simulink library "quadcopter_lib"  (R2018b)
settings: Solver=VariableStepAuto  StartTime=0.0  StopTime=10.0  RelTol=1e-3
undefined symbols (not defined in the file or in its folder): copter, grnd, IC, pos_ref
libraries: actuators_lib x1, ground_lib x1, multicopter_aerodynamics_simple_lib x1, quadcopter_propulsion_lib x1, rigidBody_lib x1
settings Model: Creator=Ybeyer  LastModifiedBy=yannic
settings SFSimCC: SimUseLocalCustomCode=off
settings RTWCC: RTWUseLocalCustomCode=off
settings CodeAppCC: StateflowObjectComments=on

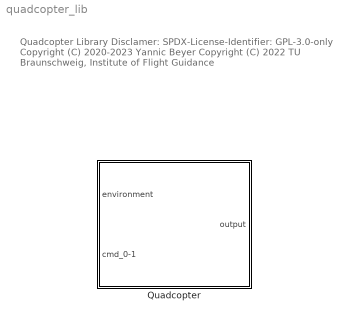
== system quadcopter_lib ==
  note: Quadcopter Library
      |
      | Disclamer:
      | SPDX-License-Identifier: GPL-3.0-only
      |
      | Copyright (C) 2020-2023 Yannic Beyer
      | Copyright (C) 2022 TU Braunschweig, Institute of Flight Guidance
  Quadcopter : Subsystem  mask{copter_=copter, IC_=IC, grnd_=grnd}
      mask prompts: copter_ "copter parameters struct"; IC_ "initial conditions struct"; grnd_ "ground contact parameters struct"
      mask DialogControl DescGroupVar Prompt: Quadcopter
      mask DialogControl DescTextVar Prompt: Standard rigid-body quadcopter model with map-based propellers and simple aerodynamics model for the frame

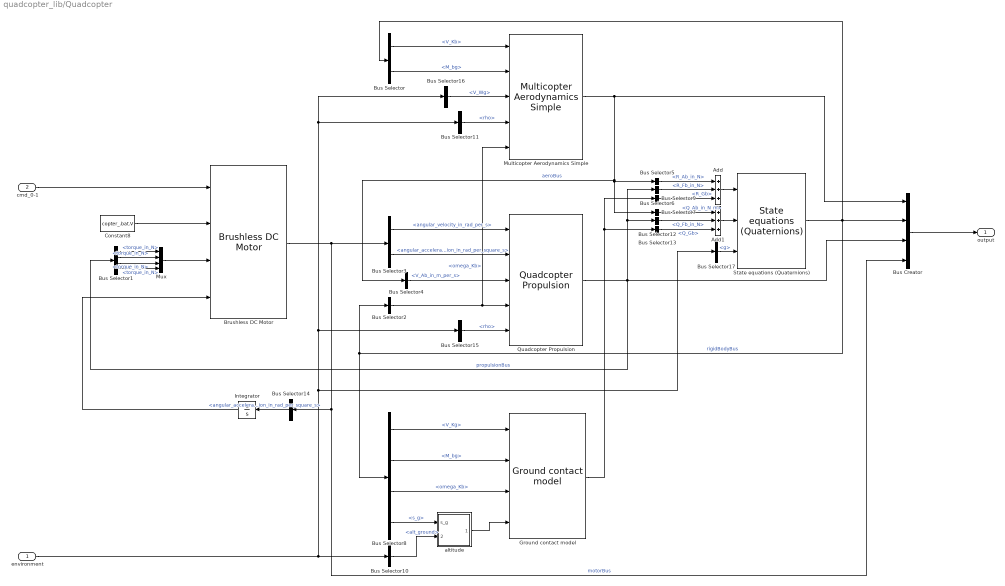
== system quadcopter_lib/Quadcopter ==
  environment : Inport  OutDataTypeStr=Bus: envirBus
  cmd_0-1 : Inport  Port=2  OutDataTypeStr=double  PortDimensions=4
  Add : Sum  Inputs=+++
  Add1 : Sum  Inputs=+++
  Brushless DC Motor : actuators_lib/Brushless DC Motor  K_T=copter_.motor.KT  J_prop=copter_.prop.I  R_i=copter_.motor.R  IC_omega=IC_.omega_mot  omega_max=Inf  omega_min=0
      settings: SourceProductName=LADAC
  Bus Creator : BusCreator  Inputs=4
  Bus Selector : BusSelector  OutputSignals=V_Kb,M_bg
  Bus Selector1 : BusSelector  OutputSignals=propeller_1.torque_in_N,propeller_2.torque_in_N,propeller_3.torque_in_N,propeller_4.torque_in_N
  Bus Selector10 : BusSelector  OutputSignals=alt_ground
  Bus Selector11 : BusSelector  OutputSignals=atmosphere.rho
  Bus Selector12 : BusSelector  OutputSignals=Q_Fb_in_N
  Bus Selector13 : BusSelector  OutputSignals=forces_and_moments.Q_Gb
  Bus Selector14 : BusSelector  OutputSignals=angular_acceleration_in_rad_per_square_s
  Bus Selector15 : BusSelector  OutputSignals=atmosphere.rho
  Bus Selector16 : BusSelector  OutputSignals=wind.V_Wg
  Bus Selector17 : BusSelector  OutputSignals=g
  Bus Selector2 : BusSelector  OutputSignals=omega_Kb
  Bus Selector3 : BusSelector  OutputSignals=angular_velocity_in_rad_per_s,angular_acceleration_in_rad_per_square_s
  Bus Selector4 : BusSelector  OutputSignals=V_Ab_in_m_per_s
  Bus Selector5 : BusSelector  OutputSignals=R_Ab_in_N
  Bus Selector6 : BusSelector  OutputSignals=R_Fb_in_N
  Bus Selector7 : BusSelector  OutputSignals=Q_Ab_in_N_m
  Bus Selector8 : BusSelector  OutputSignals=V_Kg,M_bg,omega_Kb,s_g
  Bus Selector9 : BusSelector  OutputSignals=forces_and_moments.R_Gb
  Constant8 : Constant  Value=copter_.bat.V
  Ground contact model : ground_lib/Ground contact model  m=copter_.body.m  a_max=grnd_.acc_max  xyz_c_hit=copter_.config.hitPoints_c  xyz_c_cg=copter_.config.CoG_Pos_c  ground_softness_param=grnd_.softness_parameter  k_h=grnd_.spring_stiffness  k_dot_h=grnd_.damping  mu=grnd_.friction_coef  k_V=grnd_.low_speed_friction_reduction_factor
      settings: SourceProductName=LADAC
  Integrator : Integrator  InitialCondition=IC_.omega_mot  ContinuousStateAttributes='motor_speed'
  Multicopter Aerodynamics Simple : multicopter_aerodynamics_simple_lib/Multicopter Aerodynamics Simple  copterAero=copter_.aero
      settings: SourceProductName=LADAC
  Mux : Mux
  Quadcopter Propulsion : quadcopter_propulsion_lib/Quadcopter Propulsion  copterConfig=copter_.config  map_fit=copter_.prop.map_fit  propInertia=copter_.prop.I
      settings: SourceProductName=LADAC
  State equations (Quaternions) : rigidBody_lib/State equations (Quaternions)  m=copter_.body.m  I=copter_.body.I  is_g_checked=on  g=9.81  omega_Kb_0=IC_.omega_Kb  q_bg_0=IC_.q_bg  V_Kb_0=IC_.V_Kb  s_g_0=IC_.s_Kg
      settings: SourceProductName=LADAC
  altitude : Subsystem
  output : Outport
  wires:
  Bus Selector16/1 -> Multicopter Aerodynamics Simple/3  "<V_Wg>"
  Bus Selector15/1 -> Quadcopter Propulsion/5  "<rho>"
  Bus Selector11/1 -> Multicopter Aerodynamics Simple/4  "<rho>"
  Bus Selector14/1 -> Integrator/1  "<angular_acceleration_in_rad_per_square_s>"
  environment/1 -> Bus Selector17/1, Bus Selector11/1, Bus Selector16/1, Bus Selector15/1, Bus Selector10/1
  Bus Selector2/1 -> Multicopter Aerodynamics Simple/5, Quadcopter Propulsion/4  "<omega_Kb>"
  Multicopter Aerodynamics Simple/1 -> Bus Selector4/1, Bus Selector5/1, Bus Selector7/1, Bus Creator/1  "aeroBus"
  Quadcopter Propulsion/1 -> Bus Selector6/1, Bus Selector12/1, Bus Creator/3, Bus Selector1/1  "propulsionBus"
  Bus Selector4/1 -> Quadcopter Propulsion/3  "<V_Ab_in_m_per_s>"
  State equations (Quaternions)/1 -> Bus Selector8/1, Bus Selector2/1, Bus Creator/2, Bus Selector/1  "rigidBodyBus"
  Bus Selector6/1 -> Add/2  "<R_Fb_in_N>"
  Bus Selector3/2 -> Quadcopter Propulsion/2  "<angular_acceleration_in_rad_per_square_s>"
  Bus Selector5/1 -> Add/1  "<R_Ab_in_N>"
  Bus Creator/1 -> output/1
  Brushless DC Motor/1 -> Bus Creator/4, Bus Selector14/1, Bus Selector3/1  "motorBus"
  Bus Selector9/1 -> Add/3  "<R_Gb>"
  Bus Selector8/1 -> Ground contact model/1  "<V_Kg>"
  Bus Selector8/2 -> Ground contact model/2  "<M_bg>"
  Bus Selector8/3 -> Ground contact model/3  "<omega_Kb>"
  Ground contact model/1 -> Bus Selector9/1, Bus Selector13/1
  Bus Selector1/3 -> Mux/3  "<torque_in_N>"
  Bus Selector1/1 -> Mux/1  "<torque_in_N>"
  Integrator/1 -> Brushless DC Motor/4
  Mux/1 -> Brushless DC Motor/3
  Bus Selector1/2 -> Mux/2  "<torque_in_N>"
  Bus Selector1/4 -> Mux/4  "<torque_in_N>"
  Constant8/1 -> Brushless DC Motor/2
  cmd_0-1/1 -> Brushless DC Motor/1
  Bus Selector3/1 -> Quadcopter Propulsion/1  "<angular_velocity_in_rad_per_s>"
  Add1/1 -> State equations (Quaternions)/2
  Add/1 -> State equations (Quaternions)/1
  Bus Selector7/1 -> Add1/1  "<Q_Ab_in_N_m>"
  Bus Selector12/1 -> Add1/2  "<Q_Fb_in_N>"
  Bus Selector13/1 -> Add1/3  "<Q_Gb>"
  Bus Selector8/4 -> altitude/1(s_g)  "<s_g>"
  Bus Selector10/1 -> altitude/2(h_ground)  "<alt_ground>"
  altitude/1(alt_cg) -> Ground contact model/4
  Bus Selector/2 -> Multicopter Aerodynamics Simple/2  "<M_bg>"
  Bus Selector/1 -> Multicopter Aerodynamics Simple/1  "<V_Kb>"
  Bus Selector17/1 -> State equations (Quaternions)/3  "<g>"

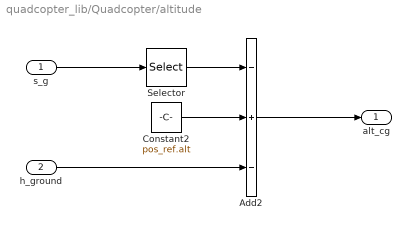
== system quadcopter_lib/Quadcopter/altitude ==
  s_g : Inport
  h_ground : Inport  Port=2
  Add2 : Sum  Inputs=-+-
  Constant2 : Constant  Value=pos_ref.alt
  Selector : Selector  InputPortWidth=3  IndexOptions=Index vector (dialog)  Indices=3  OutputSizes=1
  alt_cg : Outport
  wires:
  s_g/1 -> Selector/1
  Constant2/1 -> Add2/2
  Add2/1 -> alt_cg/1
  Selector/1 -> Add2/1
  h_ground/1 -> Add2/3
